simulink subsystem "attitude_control"  (R2025a)
settings: Solver=VariableStepAuto  StartTime=0.0  StopTime=10.0  RelTol=1e-3
values from neighbouring files (symbols this model uses):
  Kb_rate = Ki_rate    [drone_plant.m]
  Ki_rate = Kp_rate ./ facteur_Ki    [drone_plant.m]
  Kp_rate = I ./ tau    [drone_plant.m]
settings Model: Creator=flore  LastModifiedBy=flore

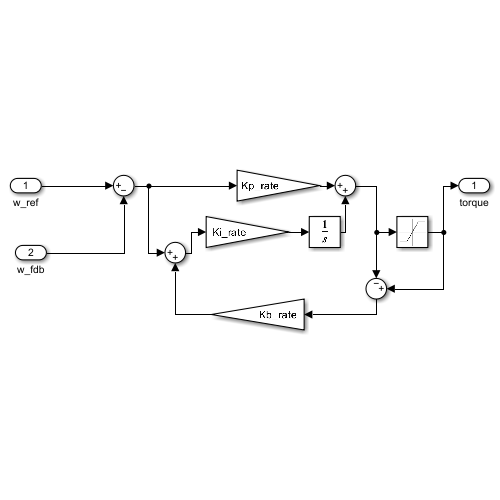
[thumbnail: Simulink's stored preview of the top-level diagram]
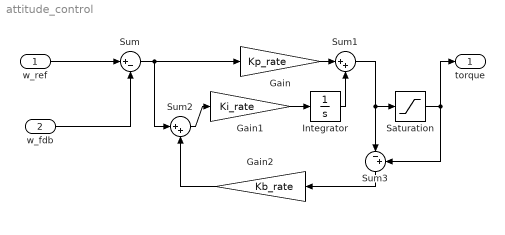
== system attitude_control ==
  w_ref : Inport
  w_fdb : Inport  Port=2
  Gain : Gain  Gain=Kp_rate
  Gain1 : Gain  Gain=Ki_rate
  Gain2 : Gain  Gain=Kb_rate
  Integrator : Integrator
  Saturation : Saturate
  Sum : Sum  Inputs=|+-
  Sum1 : Sum  Inputs=|++
  Sum2 : Sum  Inputs=|++
  Sum3 : Sum  Inputs=|-+
  torque : Outport
  wires:
  w_ref/1 -> Sum/1
  w_fdb/1 -> Sum/2
  Sum/1 -> Sum2/1, Gain/1
  Gain/1 -> Sum1/1
  Sum1/1 -> Sum3/1, Saturation/1
  Saturation/1 -> Sum3/2, torque/1
  Sum2/1 -> Gain1/1
  Sum3/1 -> Gain2/1
  Gain2/1 -> Sum2/2
  Integrator/1 -> Sum1/2
  Gain1/1 -> Integrator/1
